simulink model "ecu_safety"  (R2026a)
settings: Solver=FixedStepDiscrete  StopTime=10  FixedStep=0.001  SampleTimeConstraint=STIndependent
Description:
  | Trip decision. Source of truth for firmware/gen/ecu_safety.
settings Model: Creator=jj1001000  LastModifiedBy=jj1001000
settings OptimizationCC: DefaultUnderspecifiedDataType=single
settings DebuggingCC: ParameterPrecisionLossMsg=none
settings HardwareCC: ProdLargestAtomicInteger=Long  ProdLargestAtomicFloat=Double  ProdHWDeviceType=ARM Compatible->ARM Cortex-M
settings RTWCC: SystemTargetFile=ert.tlc  GenCodeOnly=on  Description=Embedded Coder
settings ERTTargetCC: UtilityFuncGeneration=Shared location  IncludeMdlTerminateFcn=off  CodeInterfacePackaging=Reusable function  SupportNonFinite=off

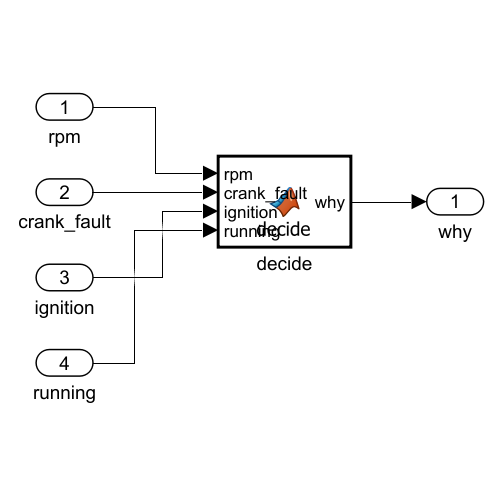
[thumbnail: Simulink's stored preview of the top-level diagram]
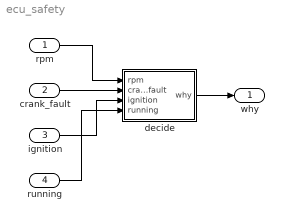
== system ecu_safety ==
  rpm : Inport  OutDataTypeStr=single
  crank_fault : Inport  Port=2  OutDataTypeStr=uint8
  ignition : Inport  Port=3  OutDataTypeStr=uint8
  running : Inport  Port=4  OutDataTypeStr=uint8
  decide : MATLAB Function  TreatAsAtomicUnit=on
  why : Outport  OutDataTypeStr=uint8
  wires:
  running/1 -> decide/4(running)
  crank_fault/1 -> decide/2(crank_fault)
  rpm/1 -> decide/1(rpm)
  ignition/1 -> decide/3(ignition)
  decide/1(why) -> why/1

== matlab function ecu_safety/decide ==
  data: rpm input single; why output uint8; crank_fault input uint8; ignition input uint8; running input uint8
function why = decide(rpm, crank_fault, ignition, running)
%#codegen
% TRIP_NONE 0, TRIP_OVERSPEED 1, TRIP_SYNC 2, TRIP_IGN 3 (safety.h)
if rpm > single(1650)
    why = uint8(1);
elseif running ~= 0 && crank_fault ~= 0
    why = uint8(2);
elseif ignition == 0
    why = uint8(3);
else
    why = uint8(0);
end
